simulink model "efficient_discrete_ADRC"  (R2025b)
settings: Solver=VariableStepAuto  StartTime=0.0  StopTime=20  RelTol=1e-3
values from neighbouring files (symbols this model uses):
  accelBC = nan(size(waypoints))    [quad_params.m]
  Alloc = [ kf,     kf,     kf,     kf ... (first row only)    [quad_params.m]
  Area = 2*L*Width    (= 0.072)    [quad_params.m]
  g = 9.81    [quad_params.m]
  h = [0 ... (first row only)    [Madgwick.m]    (also in quad_params.m = 0.2; umich_learning.m = x(:,1))
  h0 = Ts    (= 0.001)    [quad_params.m]
  h0_angle = Ts * 10    (= 0.01)    [quad_params.m]
  h0_h = Ts_h    (= 0.05)    [quad_params.m]
  inertia_mx = [Ixx; Iyy; Izz;]    [quad_params.m]
  init_h = 0.03    [quad_params.m]
  jerkBC = nan(size(waypoints))    [quad_params.m]
  K_alloc = Alloc \ diag([W, 1, 1, 1])    [quad_params.m]
  max_rad_s_2 = max_rad_s ^ 2    (= 4279618.17072)    [quad_params.m]
  r0_angle = 1000    [quad_params.m]
  r0_h = 1    [quad_params.m]
  r0_position = 1    [quad_params.m]
  rho_air = 1.225    [quad_params.m]
  rho_water = 1000    [quad_params.m]
  timePoints = [0, tTakeoff +      (0:nPerLoop*nLoops)*(tLoop/nPerLoop)]    [quad_params.m]
  Trot = 0.01    [quad_params.m]
  Ts = 0.001    [get_noise.m]    (also in quad_params.m; test.m = 0.002)
  Ts_h = 0.05    [quad_params.m]
  velBC = nan(size(waypoints))    [quad_params.m]
  W = 0.7 + 4*m_prop    (= 0.74)    [quad_params.m]
  waypoints = [0, x ... (first row only)    [quad_params.m]
undefined symbols (not defined in the file or in its folder): adrcD
libraries: eeGeneralControl x9, simulink x5, aerolibwind2 x1, shareduavrstlib x1
settings Model: Creator=David  LastModifiedBy=David

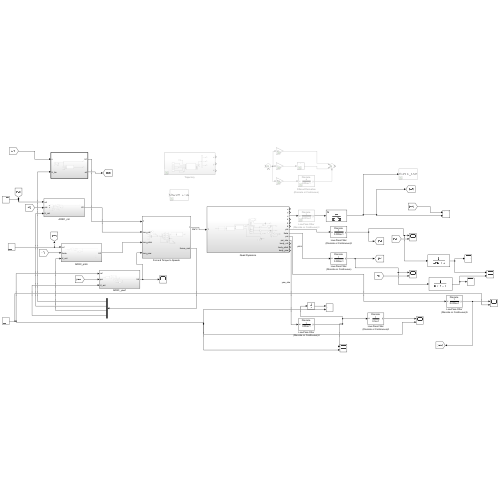
[thumbnail: Simulink's stored preview of the top-level diagram]
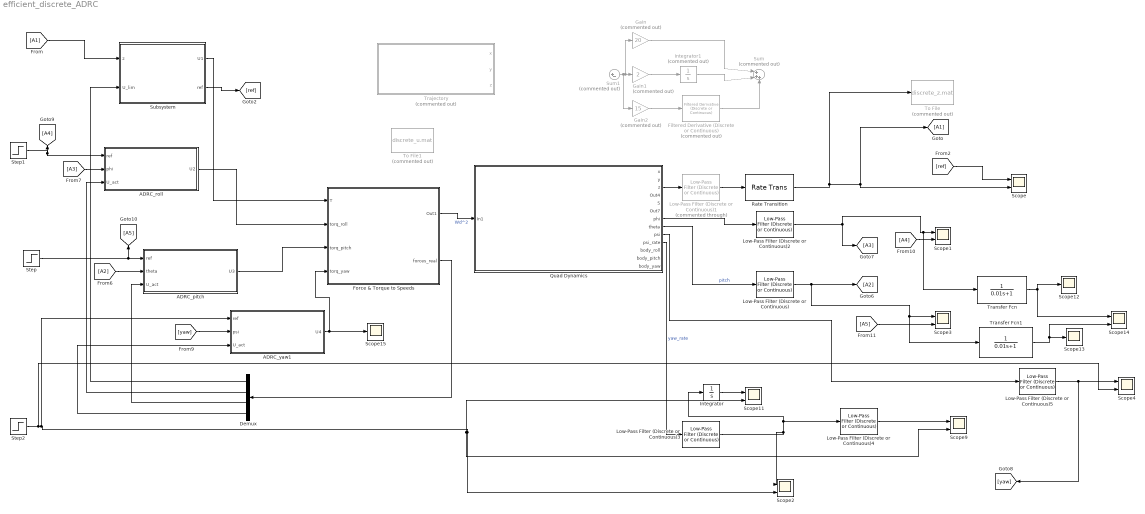
== system efficient_discrete_ADRC ==
  ADRC_pitch : Subsystem
  ADRC_roll : Subsystem
  ADRC_yaw1 : Subsystem
  Demux : Demux
  Filtered Derivative (Discrete or Continuous) : eeGeneralControl/Filtered Derivative (Discrete or Continuous)  Commented=on  K=1  T=0.05  B=inf  A=-inf  minRatio=10  init_option=Inherited from block input  x0=0  Ts=-1
      settings: LibrarySourceBlock=|
      | ee_sl_lib/General Control/Filtered Derivative
      | (Discrete or Continuous)
  Force & Torque to Speeds : Subsystem
  Gain : Gain  Commented=on  Gain=20
  Gain1 : Gain  Commented=on  Gain=2
  Gain2 : Gain  Commented=on  Gain=15
  Integrator : Integrator
  Integrator1 : Integrator  Commented=on
  Low-Pass Filter (Discrete or Continuous) : eeGeneralControl/Low-Pass Filter (Discrete or Continuous)  K=1  T=0.005  B=inf  A=-inf  init_option=Inherited from block input  x0=0  Ts=Ts
  Low-Pass Filter (Discrete or Continuous)1 : eeGeneralControl/Low-Pass Filter (Discrete or Continuous)  Commented=through  K=1  T=0.001  B=inf  A=-inf  init_option=Inherited from block input  x0=0  Ts=Ts
  Low-Pass Filter (Discrete or Continuous)2 : eeGeneralControl/Low-Pass Filter (Discrete or Continuous)  K=1  T=0.005  B=inf  A=-inf  init_option=Inherited from block input  x0=0  Ts=Ts
  Low-Pass Filter (Discrete or Continuous)3 : eeGeneralControl/Low-Pass Filter (Discrete or Continuous)  K=1  T=0.05  B=inf  A=-inf  init_option=Inherited from block input  x0=0  Ts=Ts
  Low-Pass Filter (Discrete or Continuous)4 : eeGeneralControl/Low-Pass Filter (Discrete or Continuous)  K=1  T=0.5  B=inf  A=-inf  init_option=Inherited from block input  x0=0  Ts=Ts
  Low-Pass Filter (Discrete or Continuous)5 : eeGeneralControl/Low-Pass Filter (Discrete or Continuous)  K=1  T=0.005  B=inf  A=-inf  init_option=Inherited from block input  x0=0  Ts=Ts
  Quad Dynamics : Subsystem
  Rate Transition : RateTransition  OutPortSampleTime=Ts_h
  Scope{,1..4,9,11,14} (8 alike) : Scope  NumInputPorts=2
      Scope settings: ActiveDisplayYMinimum=-0.18688766628594322  ActiveDisplayYMaximum=1.6819889965734893  DataLoggingVariableName=ScopeData2
      Scope1 settings: ActiveDisplayYMinimum=-0.13984430574300916  ActiveDisplayYMaximum=0.55327810674461919
      Scope11 settings: ActiveDisplayYMinimum=-1.1201443068824162  ActiveDisplayYMaximum=8.8240715745492686  DataLoggingVariableName=ScopeData21
      Scope14 settings: ActiveDisplayYMinimum=-0.12705190538512617  ActiveDisplayYMaximum=0.50097031332501329  DataLoggingVariableName=ScopeData29
      Scope2 settings: ActiveDisplayYMinimum=-1.0000255800633333  ActiveDisplayYMaximum=2.2551550054891538  DataLoggingVariableName=ScopeData13
      Scope3 settings: ActiveDisplayYMinimum=-1.3031757015702203  ActiveDisplayYMaximum=1.3764664599479359
      Scope4 settings: ActiveDisplayYMinimum=-0.027434331958352268  ActiveDisplayYMaximum=0.24653328293336874  DataLoggingVariableName=ScopeData4
      Scope9 settings: ActiveDisplayYMinimum=-2.6902354434565239  ActiveDisplayYMaximum=2.8491881506489021  DataLoggingVariableName=ScopeData15
  Scope12 : Scope
      settings: ActiveDisplayYMinimum=-0.051654354222600722  ActiveDisplayYMaximum=0.34551857931943891  DataLoggingVariableName=ScopeData27
  Scope13 : Scope
      settings: ActiveDisplayYMinimum=-0.043384499181721006  ActiveDisplayYMaximum=0.23881982281001995  DataLoggingVariableName=ScopeData28
  Scope15 : Scope
      settings: ActiveDisplayYMinimum=-0.42131356048161295  ActiveDisplayYMaximum=0.725418465428479  DataLoggingVariableName=ScopeData14
  Step : Step  Time=8  After=0.25  SampleTime=0
  Step1 : Step  Time=5  After=0.4  SampleTime=0
  Step2 : Step  After=0.2  SampleTime=0
  Subsystem : Subsystem  TreatAsAtomicUnit=on  SystemSampleTime=Ts_h
  Sum : Sum  Commented=on  Inputs=|+++
  Sum1 : Sum  Commented=on  Inputs=|+-
  To File : ToFile  Commented=on  Filename=discrete_z.mat  SaveFormat=Timeseries
  To File1 : ToFile  Commented=on  Filename=discrete_u.mat  SaveFormat=Timeseries
  Trajectory : Subsystem  Commented=on
  Transfer Fcn : TransferFcn  Denominator=[0.01 1]
  Transfer Fcn1 : TransferFcn  Denominator=[0.01 1]
  wires:
  Quad Dynamics/3(z) -> Low-Pass Filter (Discrete or Continuous)1/1
  [A3] -> ADRC_roll/2(phi)
  Step/1 -> ADRC_pitch/1(ref), [A5]
  Demux/2 -> ADRC_roll/3(U_act)
  Demux/4 -> ADRC_yaw1/3(U_act)
  [A5] -> Scope3/2
  [A4] -> Scope1/2
  [yaw] -> ADRC_yaw1/2(psi)
  Step1/1 -> ADRC_roll/1(ref), [A4]
  Quad Dynamics/7(phi) -> Low-Pass Filter (Discrete or Continuous)2/1
  Quad Dynamics/8(theta) -> Low-Pass Filter (Discrete or Continuous)/1  "pitch"
  Force & Torque to Speeds/1(Out1) -> Quad Dynamics/1(In1)  "Wd^2"
  Step2/1 -> Scope4/2, Scope2/2, Scope9/2, Scope11/2, ADRC_yaw1/1(ref)
  Quad Dynamics/10(psi_rate) -> Low-Pass Filter (Discrete or Continuous)3/1  "yaw_rate"
  Force & Torque to Speeds/2(forces_real) -> Demux/1
  [A2] -> ADRC_pitch/2(theta)
  Demux/3 -> ADRC_pitch/3(U_act)
  ADRC_yaw1/1(U4) -> Force & Torque to Speeds/4(torq_yaw), Scope15/1
  Integrator/1 -> Scope11/1
  Low-Pass Filter (Discrete or Continuous)1/1 -> Rate Transition/1
  Low-Pass Filter (Discrete or Continuous)2/1 -> Transfer Fcn/1, Scope1/1, [A3]
  Transfer Fcn/1 -> Scope12/1, Scope14/1
  Transfer Fcn1/1 -> Scope14/2, Scope13/1
  Low-Pass Filter (Discrete or Continuous)/1 -> Transfer Fcn1/1, Scope3/1, [A2]
  Integrator1/1 -> Sum/2
  Gain/1 -> Sum/1
  Filtered Derivative (Discrete or Continuous)/1 -> Sum/3
  Gain1/1 -> Integrator1/1
  Gain2/1 -> Filtered Derivative (Discrete or Continuous)/1
  Sum1/1 -> Gain2/1, Gain/1, Gain1/1
  [A1] -> Subsystem/1(z)
  Low-Pass Filter (Discrete or Continuous)3/1 -> Integrator/1, Low-Pass Filter (Discrete or Continuous)4/1, Scope2/1
  Low-Pass Filter (Discrete or Continuous)4/1 -> Scope9/1
  ADRC_roll/1(U2) -> Force & Torque to Speeds/2(torq_roll)
  ADRC_pitch/1(U3) -> Force & Torque to Speeds/3(torq_pitch)
  [ref] -> Scope/1
  Rate Transition/1 -> To File/1, [A1], Scope/2
  Quad Dynamics/9(psi) -> Low-Pass Filter (Discrete or Continuous)5/1
  Low-Pass Filter (Discrete or Continuous)5/1 -> [yaw], Scope4/1
  Demux/1 -> Subsystem/2(U_lim)
  Subsystem/2(ref) -> [ref]
  Subsystem/1(U1) -> Force & Torque to Speeds/1(T)

== system efficient_discrete_ADRC/ADRC_pitch ==
  ref : Inport
  theta : Inport  Port=2
  U_act : Inport  Port=3
  Constant : Constant  Value=adrcD.pitch.b0
  Divide : Product  Inputs=*/
  Filtered Derivative (Discrete or Continuous) : eeGeneralControl/Filtered Derivative (Discrete or Continuous)  K=1  T=1*Ts  B=inf  A=-inf  minRatio=1  init_option=Inherited from block input  x0=0  Ts=Ts
      settings: LibrarySourceBlock=|
      | ee_sl_lib/General Control/Filtered Derivative
      | (Discrete or Continuous)
  Gain : Gain  Gain=adrcD.pitch.k1
  Gain2 : Gain  Gain=adrcD.pitch.k2
  Scope1 : Scope
      settings: DataLoggingVariableName=ScopeData18
  Scope2 : Scope
      settings: DataLoggingVariableName=ScopeData19
  Sum1 : Sum  Inputs=|++
  Sum2 : Sum  Inputs=|++
  adrcD : Subsystem
  U3 : Outport
  wires:
  ref/1 -> Gain/1, Filtered Derivative (Discrete or Continuous)/1
  Sum1/1 -> U3/1
  Divide/1 -> Sum1/1
  Constant/1 -> Divide/2
  Gain/1 -> Sum2/1
  Filtered Derivative (Discrete or Continuous)/1 -> Gain2/1
  Gain2/1 -> Sum2/2
  Sum2/1 -> Divide/1
  adrcD/1(U) -> Sum1/2
  theta/1 -> adrcD/2(y)
  U_act/1 -> adrcD/1(U_act)

== system efficient_discrete_ADRC/ADRC_roll ==
  ref : Inport
  phi : Inport  Port=2
  U_act : Inport  Port=3
  Constant : Constant  Value=adrcD.roll.b0
  Divide : Product  Inputs=*/
  Filtered Derivative (Discrete or Continuous) : eeGeneralControl/Filtered Derivative (Discrete or Continuous)  K=1  T=1*Ts  B=inf  A=-inf  minRatio=1  init_option=Inherited from block input  x0=0  Ts=Ts
      settings: LibrarySourceBlock=|
      | ee_sl_lib/General Control/Filtered Derivative
      | (Discrete or Continuous)
  Gain : Gain  Gain=adrcD.roll.k1
  Gain2 : Gain  Gain=adrcD.roll.k2
  Scope : Scope  NumInputPorts=2
      settings: ActiveDisplayYMinimum=-0.12874999999999998  ActiveDisplayYMaximum=1.15875  DataLoggingVariableName=ScopeData3
  Scope1 : Scope  NumInputPorts=2
      settings: ActiveDisplayYMinimum=-49.999999999999986  ActiveDisplayYMaximum=450  DataLoggingVariableName=ScopeData20
  Sum1 : Sum  Inputs=|++
  Sum2 : Sum  Inputs=|++
  TD1 : Subsystem
  adrcD : Subsystem
  U2 : Outport
  wires:
  ref/1 -> Filtered Derivative (Discrete or Continuous)/1, Scope/2, TD1/1(v)
  Sum1/1 -> U2/1
  Divide/1 -> Sum1/1
  Constant/1 -> Divide/2
  Gain/1 -> Sum2/1
  TD1/2(dref) -> Scope/1, Scope1/2, Gain2/1
  Gain2/1 -> Sum2/2
  Sum2/1 -> Divide/1
  adrcD/1(U) -> Sum1/2
  U_act/1 -> adrcD/1(U_act)
  phi/1 -> adrcD/2(y)
  TD1/1(ref) -> Gain/1
  Filtered Derivative (Discrete or Continuous)/1 -> Scope1/1

== system efficient_discrete_ADRC/ADRC_yaw1 ==
  ref : Inport
  psi : Inport  Port=2
  U_act : Inport  Port=3
  Constant : Constant  Value=adrcD.yaw.b0
  Divide : Product  Inputs=*/
  Gain : Gain  Gain=adrcD.yaw.k1
  Gain2 : Gain  Gain=adrcD.yaw.k2
  Scope : Scope
      settings: DataLoggingVariableName=ScopeData23
  Sum1 : Sum  Inputs=|++
  Sum2 : Sum  Inputs=|++
  TD1 : Subsystem
  adrcD : Subsystem
  U4 : Outport
  wires:
  Sum1/1 -> U4/1
  Divide/1 -> Sum1/1
  Constant/1 -> Divide/2
  ref/1 -> TD1/1(v)
  TD1/1(ref) -> Gain/1
  TD1/2(dref) -> Gain2/1
  Gain/1 -> Sum2/1
  Gain2/1 -> Sum2/2
  Sum2/1 -> Scope/1, Divide/1
  adrcD/1(U) -> Sum1/2
  U_act/1 -> adrcD/1(U_act)
  psi/1 -> adrcD/2(y)

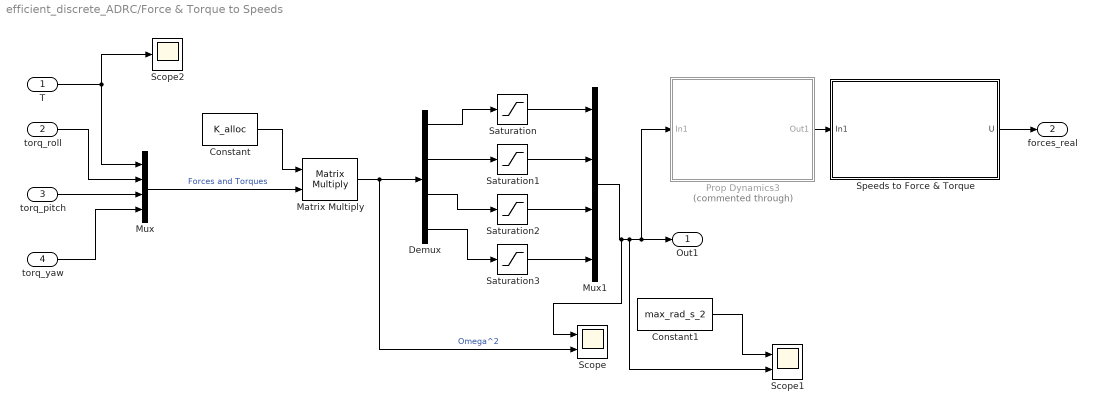
== system efficient_discrete_ADRC/Force & Torque to Speeds ==
  T : Inport
  torq_roll : Inport  Port=2
  torq_pitch : Inport  Port=3
  torq_yaw : Inport  Port=4
  Constant : Constant  Value=K_alloc
  Constant1 : Constant  Value=max_rad_s_2
  Demux : Demux
  Matrix Multiply : Product  Multiplication=Matrix(*)
  Mux : Mux
  Mux1 : Mux
  Prop Dynamics3 : Subsystem  Commented=through
  Saturation{,1..3} (4 alike) : Saturate  UpperLimit=max_rad_s_2  LowerLimit=0
  Scope : Scope  NumInputPorts=2
      settings: ActiveDisplayYMinimum=-2.4803736586129647E+6  ActiveDisplayYMaximum=5.5202696731347125E+6  DataLoggingVariableName=ScopeData11
  Scope1 : Scope  NumInputPorts=2
      settings: ActiveDisplayYMinimum=-534952.27133938007  ActiveDisplayYMaximum=4.8145704420544216E+6  DataLoggingVariableName=ScopeData25
  Scope2 : Scope
      settings: ActiveDisplayYMinimum=-22.315254964417129  ActiveDisplayYMaximum=34.792796764645914  DataLoggingVariableName=ScopeData9
  Speeds to Force & Torque : Subsystem
  Out1 : Outport
  forces_real : Outport  Port=2
  wires:
  Matrix Multiply/1 -> Scope/2, Demux/1  "Omega^2"
  torq_yaw/1 -> Mux/4
  torq_pitch/1 -> Mux/3
  torq_roll/1 -> Mux/2
  T/1 -> Mux/1, Scope2/1
  Constant/1 -> Matrix Multiply/1
  Mux/1 -> Matrix Multiply/2  "Forces and Torques"
  Saturation3/1 -> Mux1/4
  Demux/4 -> Saturation3/1
  Demux/2 -> Saturation1/1
  Demux/1 -> Saturation/1
  Demux/3 -> Saturation2/1
  Saturation1/1 -> Mux1/2
  Saturation/1 -> Mux1/1
  Saturation2/1 -> Mux1/3
  Mux1/1 -> Scope/1, Scope1/2, Prop Dynamics3/1(In1), Out1/1
  Speeds to Force & Torque/1(U) -> forces_real/1
  Prop Dynamics3/1(Out1) -> Speeds to Force & Torque/1(In1)
  Constant1/1 -> Scope1/1

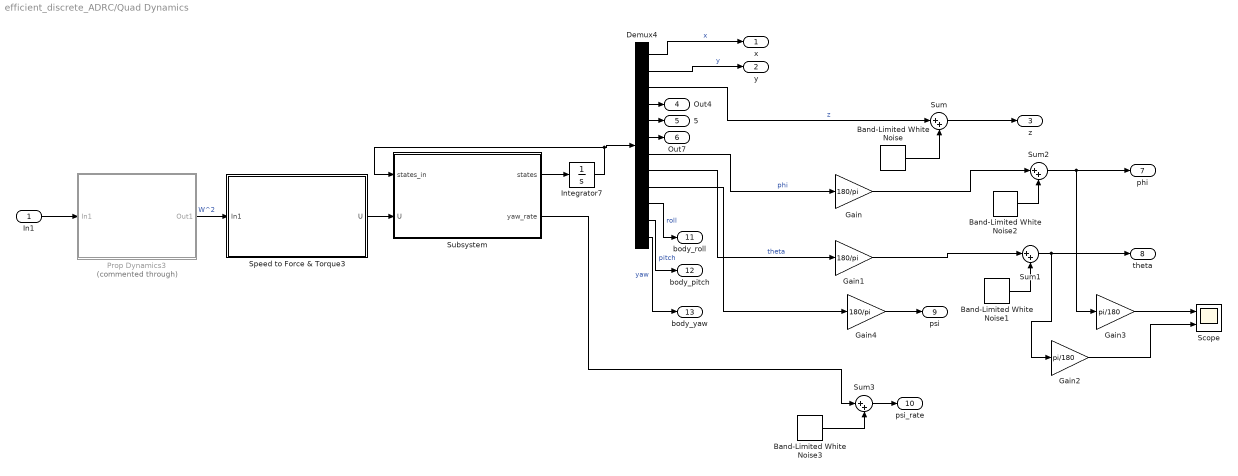
== system efficient_discrete_ADRC/Quad Dynamics ==
  In1 : Inport
  Band-Limited White Noise : simulink/Sources/Band-Limited White Noise  Cov=[2.6540e-06]  Ts=Ts_h  seed=[23341]
  Band-Limited White Noise1 : simulink/Sources/Band-Limited White Noise  Cov=[2e-6]  Ts=0.001  seed=[23342]
  Band-Limited White Noise2 : simulink/Sources/Band-Limited White Noise  Cov=[2e-6]  Ts=0.001  seed=[23341]
  Band-Limited White Noise3 : simulink/Sources/Band-Limited White Noise  Cov=[3.7430331138e-5]  Ts=0.001  seed=[23343]
  Demux4 : Demux  Outputs=12
  Gain : Gain  Gain=180/pi
  Gain1 : Gain  Gain=180/pi
  Gain2 : Gain  Gain=pi/180
  Gain3 : Gain  Gain=pi/180
  Gain4 : Gain  Gain=180/pi
  Integrator7 : Integrator  InitialCondition=zeros(12,1)
  Prop Dynamics3 : Subsystem  Commented=through
  Scope : Scope  NumInputPorts=2
      settings: ActiveDisplayYMinimum=-1  ActiveDisplayYMaximum=1  DataLoggingVariableName=ScopeData16
  Speed to Force & Torque3 : Subsystem
  Subsystem : Subsystem
  Sum{,1..3} (4 alike) : Sum  Inputs=|++
  x : Outport
  y : Outport  Port=2
  z : Outport  Port=3
  Out4 : Outport  Port=4
  5 : Outport  Port=5
  Out7 : Outport  Port=6
  phi : Outport  Port=7
  theta : Outport  Port=8
  psi : Outport  Port=9
  psi_rate : Outport  Port=10
  body_roll : Outport  Port=11
  body_pitch : Outport  Port=12
  body_yaw : Outport  Port=13
  wires:
  Demux4/2 -> y/1  "y"
  Prop Dynamics3/1(Out1) -> Speed to Force & Torque3/1(In1)  "W^2"
  Demux4/1 -> x/1  "x"
  Subsystem/1(states) -> Integrator7/1
  Speed to Force & Torque3/1(U) -> Subsystem/2(U)
  Integrator7/1 -> Demux4/1, Subsystem/1(states_in)
  Demux4/10 -> body_roll/1  "roll"
  Demux4/7 -> Gain/1  "phi"
  Demux4/3 -> Sum/1  "z"
  Demux4/8 -> Gain1/1  "theta"
  Demux4/11 -> body_pitch/1  "pitch"
  Demux4/12 -> body_yaw/1  "yaw"
  Demux4/6 -> Out7/1
  Demux4/5 -> 5/1
  Demux4/4 -> Out4/1
  In1/1 -> Prop Dynamics3/1(In1)
  Subsystem/2(yaw_rate) -> Sum3/1
  Sum/1 -> z/1
  Band-Limited White Noise/1 -> Sum/2
  Band-Limited White Noise1/1 -> Sum1/2
  Sum1/1 -> Gain2/1, theta/1
  Band-Limited White Noise2/1 -> Sum2/2
  Sum2/1 -> Gain3/1, phi/1
  Band-Limited White Noise3/1 -> Sum3/2
  Sum3/1 -> psi_rate/1
  Gain/1 -> Sum2/1
  Gain1/1 -> Sum1/1
  Gain3/1 -> Scope/1
  Gain2/1 -> Scope/2
  Demux4/9 -> Gain4/1
  Gain4/1 -> psi/1

== system efficient_discrete_ADRC/Subsystem ==
  z : Inport
  U_lim : Inport  Port=2
  ADRC_z : Subsystem
  Constant4 : Constant  Value=init_h
  Step3 : Step  Time=2
  Sum7 : Sum  Inputs=|++
  U1 : Outport
  ref : Outport  Port=2
  wires:
  Sum7/1 -> ADRC_z/1(ref), ref/1  "ref"
  Step3/1 -> Sum7/1  "v"
  U_lim/1 -> ADRC_z/3(U_lim)
  ADRC_z/1(U1) -> U1/1
  Constant4/1 -> Sum7/2
  z/1 -> ADRC_z/2(z)

== system efficient_discrete_ADRC/Trajectory ==
  Constant1 : Constant  Value=timePoints
  Constant2 : Constant  Value=waypoints
  Constant3 : Constant  Value=velBC
  Constant4 : Constant  Value=accelBC
  Constant5 : Constant  Value=jerkBC
  Demux : Demux  Outputs=3
  Minimum Jerk Polynomial Trajectory : shareduavrstlib/Minimum Jerk Polynomial Trajectory  ShowBCInputPort=on  ShowPolynomialCoefs=off  ShowStatusOutputPort=off  TimeAllocation=off  TimeWeight=100  MinSegmentTime=0.1  MaxSegmentTime=1  MaxIteration=1500  MaxTime=10  SimulateUsing=Interpreted execution
  Ramp : simulink/Sources/Ramp  slope=1  start=0  InitialOutput=0
  Scope8 : Scope
      settings: ActiveDisplayYMinimum=-1  ActiveDisplayYMaximum=1  DataLoggingVariableName=ScopeData17
  Terminator : Terminator
  Terminator1 : Terminator
  Terminator2 : Terminator
  x : Outport
  y : Outport  Port=2
  z : Outport  Port=3
  wires:
  Minimum Jerk Polynomial Trajectory/4 -> Terminator1/1
  Minimum Jerk Polynomial Trajectory/2 -> Scope8/1
  Constant3/1 -> Minimum Jerk Polynomial Trajectory/4
  Constant2/1 -> Minimum Jerk Polynomial Trajectory/2
  Ramp/1 -> Minimum Jerk Polynomial Trajectory/1
  Minimum Jerk Polynomial Trajectory/3 -> Terminator/1
  Constant5/1 -> Minimum Jerk Polynomial Trajectory/6
  Constant4/1 -> Minimum Jerk Polynomial Trajectory/5
  Minimum Jerk Polynomial Trajectory/5 -> Terminator2/1
  Constant1/1 -> Minimum Jerk Polynomial Trajectory/3
  Minimum Jerk Polynomial Trajectory/1 -> Demux/1  "height"
  Demux/1 -> x/1
  Demux/2 -> y/1
  Demux/3 -> z/1

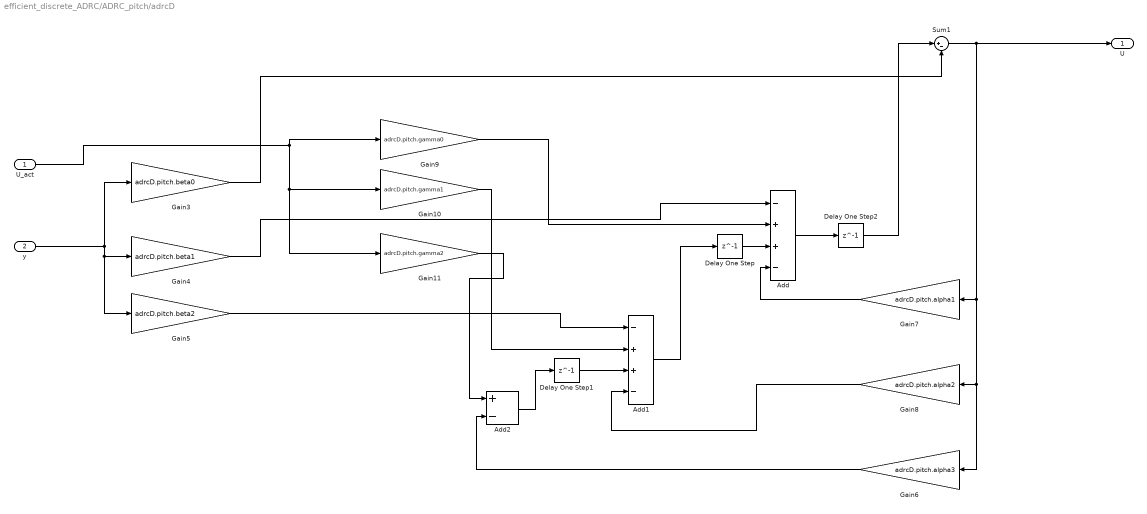
== system efficient_discrete_ADRC/ADRC_pitch/adrcD ==
  U_act : Inport
  y : Inport  Port=2
  Add : Sum  Inputs=-++-
  Add1 : Sum  Inputs=-++-
  Add2 : Sum  Inputs=+-
  Delay One Step : Delay  DelayLength=1  SampleTime=Ts
  Delay One Step1 : Delay  DelayLength=1  SampleTime=Ts
  Delay One Step2 : Delay  DelayLength=1  SampleTime=Ts
  Gain10 : Gain  Gain=adrcD.pitch.gamma1
  Gain11 : Gain  Gain=adrcD.pitch.gamma2
  Gain3 : Gain  Gain=adrcD.pitch.beta0
  Gain4 : Gain  Gain=adrcD.pitch.beta1
  Gain5 : Gain  Gain=adrcD.pitch.beta2
  Gain6 : Gain  Gain=adrcD.pitch.alpha3
  Gain7 : Gain  Gain=adrcD.pitch.alpha1
  Gain8 : Gain  Gain=adrcD.pitch.alpha2
  Gain9 : Gain  Gain=adrcD.pitch.gamma0
  Sum1 : Sum  Inputs=|+-
  U : Outport
  wires:
  Gain4/1 -> Add/1
  Gain8/1 -> Add1/4
  Add2/1 -> Delay One Step1/1
  y/1 -> Gain5/1, Gain4/1, Gain3/1
  U_act/1 -> Gain9/1, Gain11/1, Gain10/1
  Gain7/1 -> Add/4
  Gain11/1 -> Add2/1
  Gain3/1 -> Sum1/2
  Sum1/1 -> U/1, Gain6/1, Gain8/1, Gain7/1
  Add1/1 -> Delay One Step/1
  Gain5/1 -> Add1/1
  Gain10/1 -> Add1/2
  Add/1 -> Delay One Step2/1
  Gain9/1 -> Add/2
  Delay One Step1/1 -> Add1/3
  Delay One Step2/1 -> Sum1/1
  Gain6/1 -> Add2/2
  Delay One Step/1 -> Add/3

== system efficient_discrete_ADRC/ADRC_roll/TD1 ==
  v : Inport
  Constant11 : Constant  Value=r0_angle
  Constant12 : Constant  Value=h0_angle
  Delay One Step : Delay  DelayLength=1  SampleTime=Ts
  Delay One Step1 : Delay  DelayLength=1  SampleTime=Ts
  Gain3 : Gain  Gain=Ts
  Gain4 : Gain  Gain=Ts
  Sum1 : Sum  Inputs=|++
  Sum6 : Sum  Inputs=|++
  Sum7 : Sum  Inputs=|+-
  fhan : MATLAB Function  TreatAsAtomicUnit=on
  ref : Outport
  dref : Outport  Port=2
  wires:
  v/1 -> Sum7/2
  Constant12/1 -> fhan/4(h0)
  Sum7/1 -> fhan/1(e)
  Constant11/1 -> fhan/3(r0)
  Delay One Step1/1 -> fhan/2(v2), Sum6/2, Gain4/1  "v2(k)"
  Gain4/1 -> Sum1/2
  Sum1/1 -> ref/1, Delay One Step/1  "v1(k+1)"
  Sum6/1 -> dref/1, Delay One Step1/1  "v2(k+1)"
  Gain3/1 -> Sum6/1
  Delay One Step/1 -> Sum1/1, Sum7/1  "v1"
  fhan/1(u) -> Gain3/1

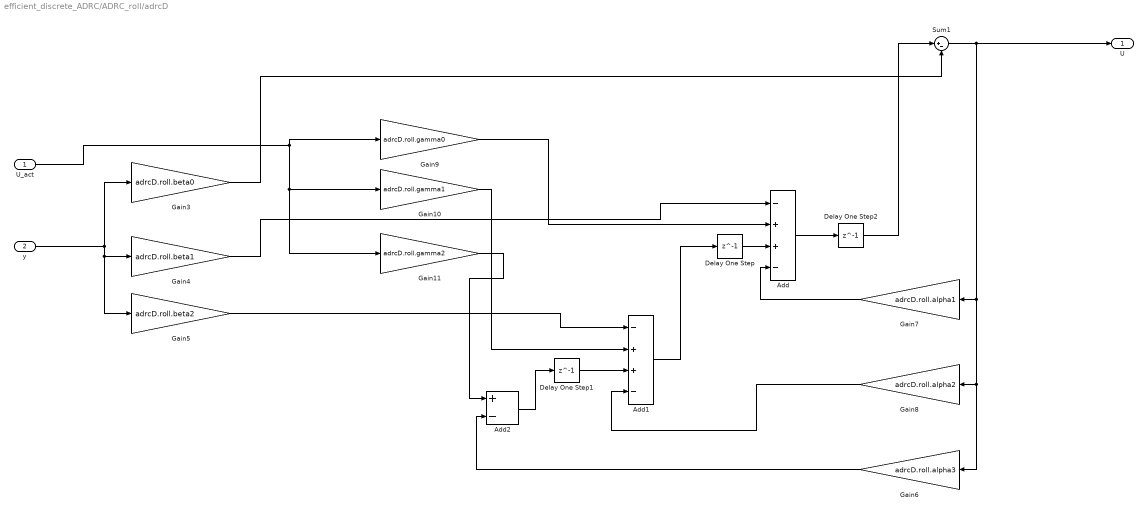
== system efficient_discrete_ADRC/ADRC_roll/adrcD ==
  U_act : Inport
  y : Inport  Port=2
  Add : Sum  Inputs=-++-
  Add1 : Sum  Inputs=-++-
  Add2 : Sum  Inputs=+-
  Delay One Step : Delay  DelayLength=1  SampleTime=Ts
  Delay One Step1 : Delay  DelayLength=1  SampleTime=Ts
  Delay One Step2 : Delay  DelayLength=1  SampleTime=Ts
  Gain10 : Gain  Gain=adrcD.roll.gamma1
  Gain11 : Gain  Gain=adrcD.roll.gamma2
  Gain3 : Gain  Gain=adrcD.roll.beta0
  Gain4 : Gain  Gain=adrcD.roll.beta1
  Gain5 : Gain  Gain=adrcD.roll.beta2
  Gain6 : Gain  Gain=adrcD.roll.alpha3
  Gain7 : Gain  Gain=adrcD.roll.alpha1
  Gain8 : Gain  Gain=adrcD.roll.alpha2
  Gain9 : Gain  Gain=adrcD.roll.gamma0
  Sum1 : Sum  Inputs=|+-
  U : Outport
  wires:
  Gain4/1 -> Add/1
  Gain8/1 -> Add1/4
  Add2/1 -> Delay One Step1/1
  y/1 -> Gain5/1, Gain4/1, Gain3/1
  U_act/1 -> Gain9/1, Gain11/1, Gain10/1
  Gain7/1 -> Add/4
  Gain11/1 -> Add2/1
  Gain3/1 -> Sum1/2
  Sum1/1 -> U/1, Gain6/1, Gain8/1, Gain7/1
  Add1/1 -> Delay One Step/1
  Gain5/1 -> Add1/1
  Gain10/1 -> Add1/2
  Add/1 -> Delay One Step2/1
  Gain9/1 -> Add/2
  Delay One Step1/1 -> Add1/3
  Delay One Step2/1 -> Sum1/1
  Gain6/1 -> Add2/2
  Delay One Step/1 -> Add/3

== system efficient_discrete_ADRC/ADRC_yaw1/TD1 ==
  v : Inport
  Constant11 : Constant  Value=r0_position
  Constant12 : Constant  Value=h0
  Delay One Step : Delay  DelayLength=1  SampleTime=Ts
  Delay One Step1 : Delay  DelayLength=1  SampleTime=Ts
  Gain3 : Gain  Gain=Ts
  Gain4 : Gain  Gain=Ts
  Sum1 : Sum  Inputs=|++
  Sum6 : Sum  Inputs=|++
  Sum7 : Sum  Inputs=|+-
  fhan : MATLAB Function  TreatAsAtomicUnit=on
  ref : Outport
  dref : Outport  Port=2
  wires:
  v/1 -> Sum7/2
  Constant12/1 -> fhan/4(h0)
  Sum7/1 -> fhan/1(e)
  Constant11/1 -> fhan/3(r0)
  Delay One Step1/1 -> fhan/2(v2), Sum6/2, Gain4/1  "v2(k)"
  Gain4/1 -> Sum1/2
  Sum1/1 -> ref/1, Delay One Step/1  "v1(k+1)"
  Sum6/1 -> dref/1, Delay One Step1/1  "v2(k+1)"
  Gain3/1 -> Sum6/1
  Delay One Step/1 -> Sum1/1, Sum7/1  "v1"
  fhan/1(u) -> Gain3/1

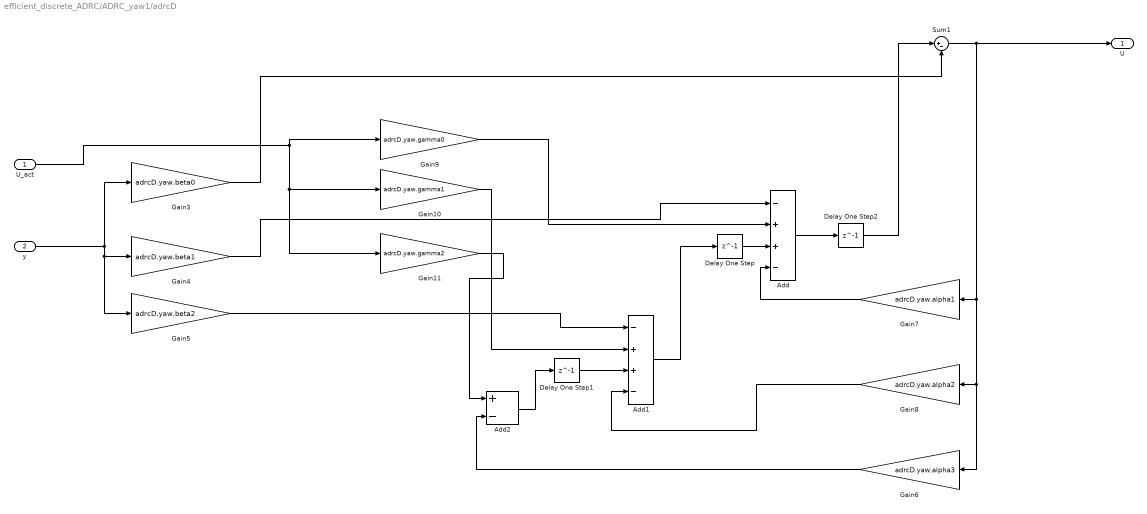
== system efficient_discrete_ADRC/ADRC_yaw1/adrcD ==
  U_act : Inport
  y : Inport  Port=2
  Add : Sum  Inputs=-++-
  Add1 : Sum  Inputs=-++-
  Add2 : Sum  Inputs=+-
  Delay One Step : Delay  DelayLength=1  SampleTime=Ts
  Delay One Step1 : Delay  DelayLength=1  SampleTime=Ts
  Delay One Step2 : Delay  DelayLength=1  SampleTime=Ts
  Gain10 : Gain  Gain=adrcD.yaw.gamma1
  Gain11 : Gain  Gain=adrcD.yaw.gamma2
  Gain3 : Gain  Gain=adrcD.yaw.beta0
  Gain4 : Gain  Gain=adrcD.yaw.beta1
  Gain5 : Gain  Gain=adrcD.yaw.beta2
  Gain6 : Gain  Gain=adrcD.yaw.alpha3
  Gain7 : Gain  Gain=adrcD.yaw.alpha1
  Gain8 : Gain  Gain=adrcD.yaw.alpha2
  Gain9 : Gain  Gain=adrcD.yaw.gamma0
  Sum1 : Sum  Inputs=|+-
  U : Outport
  wires:
  Gain4/1 -> Add/1
  Gain8/1 -> Add1/4
  Add2/1 -> Delay One Step1/1
  y/1 -> Gain5/1, Gain4/1, Gain3/1
  U_act/1 -> Gain9/1, Gain11/1, Gain10/1
  Gain7/1 -> Add/4
  Gain11/1 -> Add2/1
  Gain3/1 -> Sum1/2
  Sum1/1 -> U/1, Gain6/1, Gain8/1, Gain7/1
  Add1/1 -> Delay One Step/1
  Gain5/1 -> Add1/1
  Gain10/1 -> Add1/2
  Add/1 -> Delay One Step2/1
  Gain9/1 -> Add/2
  Delay One Step1/1 -> Add1/3
  Delay One Step2/1 -> Sum1/1
  Gain6/1 -> Add2/2
  Delay One Step/1 -> Add/3

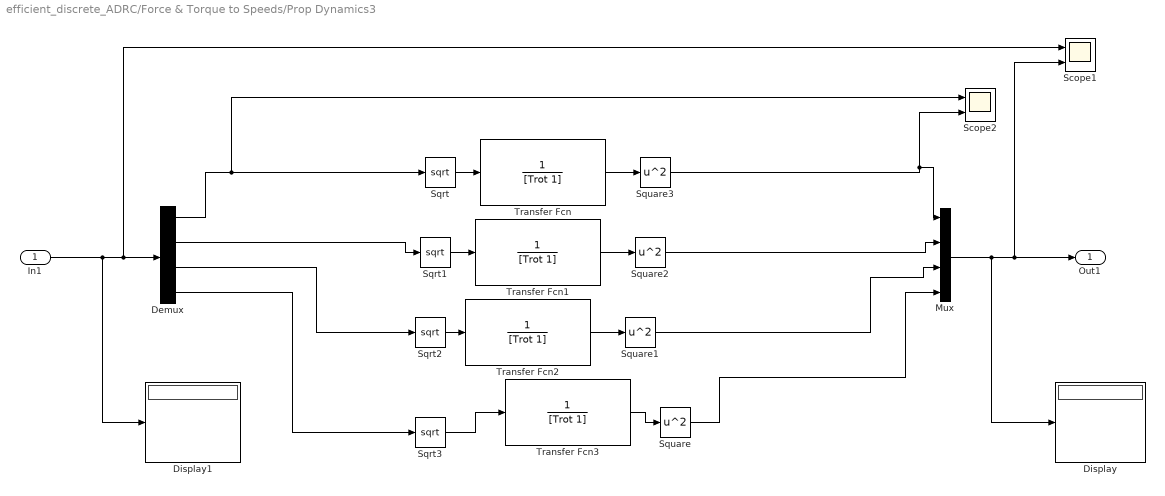
== system efficient_discrete_ADRC/Force & Torque to Speeds/Prop Dynamics3 ==
  In1 : Inport
  Demux : Demux
  Display : Display
  Display1 : Display
  Mux : Mux
  Scope1 : Scope  NumInputPorts=2
      settings: ActiveDisplayYMinimum=112181.7837613984  ActiveDisplayYMaximum=826252.36344831332  DataLoggingVariableName=ScopeData22
  Scope2 : Scope  NumInputPorts=2
      settings: ActiveDisplayYMinimum=474145.79333634069  ActiveDisplayYMaximum=566090.11578068486  DataLoggingVariableName=ScopeData26
  Sqrt{,1..3} (4 alike) : Sqrt
  Square{,1..3} (4 alike) : Math  Operator=square
  Transfer Fcn{,1..3} (4 alike) : TransferFcn  Denominator=[Trot 1]
  Out1 : Outport
  wires:
  Square/1 -> Mux/4
  Demux/4 -> Sqrt3/1
  Demux/3 -> Sqrt2/1
  Demux/2 -> Sqrt1/1
  Demux/1 -> Sqrt/1, Scope2/1
  Sqrt3/1 -> Transfer Fcn3/1
  Sqrt2/1 -> Transfer Fcn2/1
  Sqrt1/1 -> Transfer Fcn1/1
  Sqrt/1 -> Transfer Fcn/1
  Transfer Fcn3/1 -> Square/1
  Transfer Fcn2/1 -> Square1/1
  Transfer Fcn/1 -> Square3/1
  Transfer Fcn1/1 -> Square2/1
  Mux/1 -> Scope1/2, Out1/1, Display/1
  In1/1 -> Scope1/1, Demux/1, Display1/1
  Square3/1 -> Scope2/2, Mux/1
  Square2/1 -> Mux/2
  Square1/1 -> Mux/3

== system efficient_discrete_ADRC/Force & Torque to Speeds/Speeds to Force & Torque ==
  In1 : Inport
  Constant1 : Constant  Value=Alloc
  Matrix Multiply1 : Product  Multiplication=Matrix(*)
  U : Outport
  wires:
  Constant1/1 -> Matrix Multiply1/1
  Matrix Multiply1/1 -> U/1
  In1/1 -> Matrix Multiply1/2  "Omega^2"

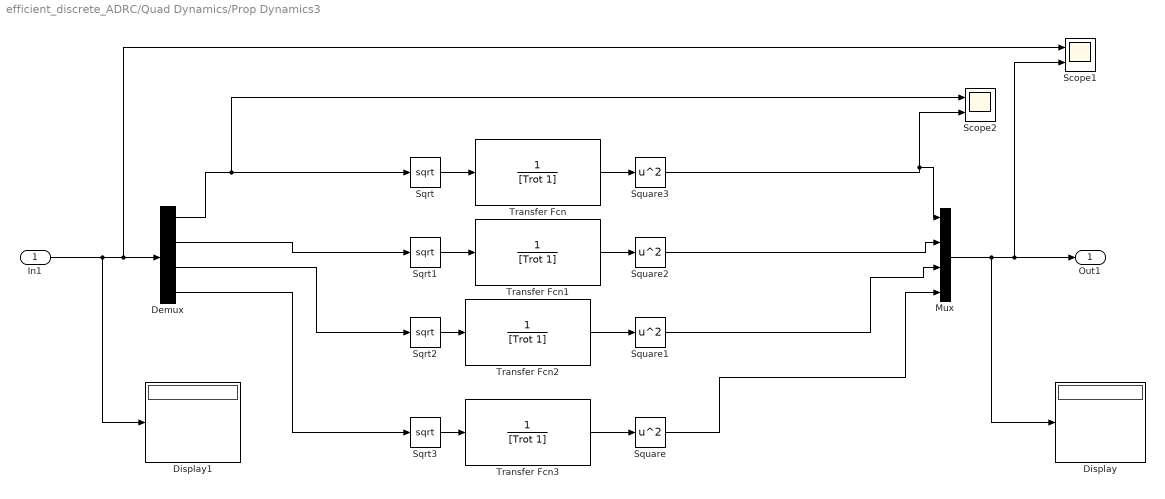
== system efficient_discrete_ADRC/Quad Dynamics/Prop Dynamics3 ==
  In1 : Inport
  Demux : Demux
  Display : Display
  Display1 : Display
  Mux : Mux
  Scope1 : Scope  NumInputPorts=2
      settings: ActiveDisplayYMinimum=-75977.2512965213  ActiveDisplayYMaximum=683795.26166869176  DataLoggingVariableName=ScopeData22
  Scope2 : Scope  NumInputPorts=2
      settings: ActiveDisplayYMinimum=-75859.286983978411  ActiveDisplayYMaximum=682733.58285580587  DataLoggingVariableName=ScopeData26
  Sqrt{,1..3} (4 alike) : Sqrt
  Square{,1..3} (4 alike) : Math  Operator=square
  Transfer Fcn{,1..3} (4 alike) : TransferFcn  Denominator=[Trot 1]
  Out1 : Outport
  wires:
  Square/1 -> Mux/4
  Demux/4 -> Sqrt3/1
  Demux/3 -> Sqrt2/1
  Demux/2 -> Sqrt1/1
  Demux/1 -> Sqrt/1, Scope2/1
  Sqrt3/1 -> Transfer Fcn3/1
  Sqrt2/1 -> Transfer Fcn2/1
  Sqrt1/1 -> Transfer Fcn1/1
  Sqrt/1 -> Transfer Fcn/1
  Transfer Fcn3/1 -> Square/1
  Transfer Fcn2/1 -> Square1/1
  Transfer Fcn/1 -> Square3/1
  Transfer Fcn1/1 -> Square2/1
  Mux/1 -> Scope1/2, Out1/1, Display/1
  In1/1 -> Scope1/1, Demux/1, Display1/1
  Square3/1 -> Scope2/2, Mux/1
  Square2/1 -> Mux/2
  Square1/1 -> Mux/3

== system efficient_discrete_ADRC/Quad Dynamics/Speed to Force & Torque3 ==
  In1 : Inport
  Constant1 : Constant  Value=Alloc
  Matrix Multiply1 : Product  Multiplication=Matrix(*)
  U : Outport
  wires:
  Constant1/1 -> Matrix Multiply1/1
  Matrix Multiply1/1 -> U/1
  In1/1 -> Matrix Multiply1/2  "Omega^2"

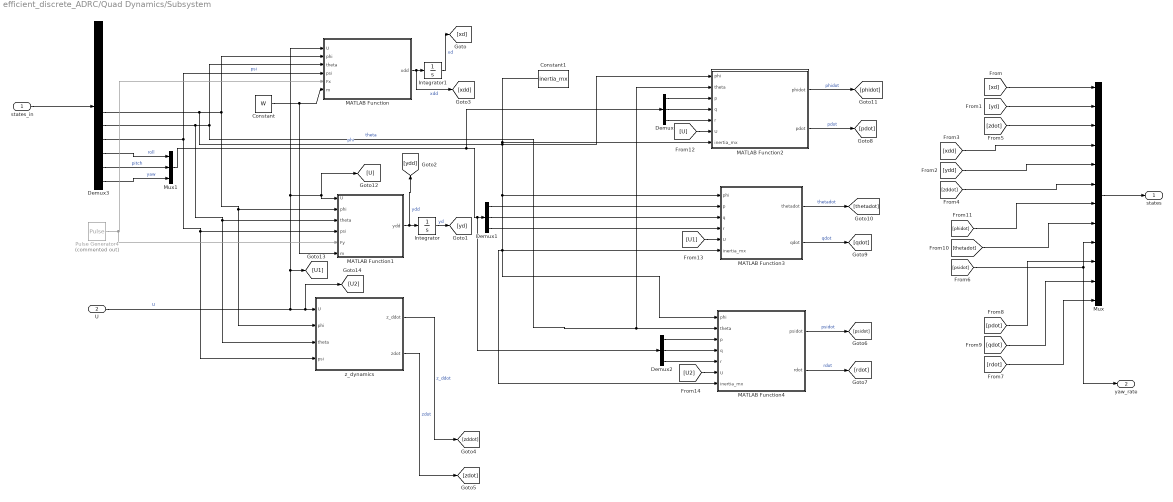
== system efficient_discrete_ADRC/Quad Dynamics/Subsystem ==
  states_in : Inport
  U : Inport  Port=2
  Constant : Constant  Value=W
  Constant1 : Constant  Value=inertia_mx
  Demux : Demux  Outputs=3
  Demux1 : Demux  Outputs=3
  Demux2 : Demux  Outputs=3
  Demux3 : Demux  Outputs=12
  Integrator : Integrator
  Integrator1 : Integrator
  MATLAB Function : MATLAB Function  TreatAsAtomicUnit=on
  MATLAB Function1 : MATLAB Function  TreatAsAtomicUnit=on
  MATLAB Function2 : MATLAB Function  TreatAsAtomicUnit=on
  MATLAB Function3 : MATLAB Function  TreatAsAtomicUnit=on
  MATLAB Function4 : MATLAB Function  TreatAsAtomicUnit=on
  Mux : Mux  Inputs=12
  Mux1 : Mux  Inputs=3
  Pulse Generator4 : DiscretePulseGenerator  Commented=on  PulseType=Time based  Amplitude=0.1  Period=5  PulseWidth=30  PhaseDelay=6
  z_dynamics : Subsystem
  states : Outport
  yaw_rate : Outport  Port=2
  wires:
  MATLAB Function/1(xdd) -> [xdd], Integrator1/1  "xdd"
  MATLAB Function1/1(ydd) -> [ydd], Integrator/1  "ydd"
  Mux/1 -> states/1
  states_in/1 -> Demux3/1
  U/1 -> [U2], z_dynamics/1(U), MATLAB Function/1(U), [U], MATLAB Function1/1(U), [U1]  "U"
  Demux3/7 -> MATLAB Function3/1(phi), MATLAB Function4/1(phi), MATLAB Function2/1(phi), MATLAB Function/2(phi), z_dynamics/2(phi), MATLAB Function1/2(phi)  "phi"
  Demux3/8 -> z_dynamics/3(theta), MATLAB Function1/3(theta), MATLAB Function2/2(theta), MATLAB Function4/2(theta), MATLAB Function/3(theta)  "theta"
  Demux3/9 -> z_dynamics/4(psi), MATLAB Function1/4(psi), MATLAB Function/4(psi)  "psi"
  Constant/1 -> MATLAB Function/6(m), MATLAB Function1/6(m)
  Constant1/1 -> MATLAB Function4/7(inertia_mx), MATLAB Function3/6(inertia_mx), MATLAB Function2/7(inertia_mx)
  Demux3/11 -> Mux1/2  "pitch"
  Demux3/12 -> Mux1/3  "yaw"
  Demux3/10 -> Mux1/1  "roll"
  Mux1/1 -> Demux/1, Demux2/1, Demux1/1
  Demux1/1 -> MATLAB Function3/2(p)
  Demux1/2 -> MATLAB Function3/3(q)
  Demux1/3 -> MATLAB Function3/4(r)
  Demux2/1 -> MATLAB Function4/3(p)
  Demux2/2 -> MATLAB Function4/4(q)
  Demux2/3 -> MATLAB Function4/5(r)
  Demux/1 -> MATLAB Function2/3(p)
  Demux/2 -> MATLAB Function2/4(q)
  Demux/3 -> MATLAB Function2/5(r)
  Integrator1/1 -> [xd]  "xd"
  [xd] -> Mux/1
  Integrator/1 -> [yd]  "yd"
  [yd] -> Mux/2
  [ydd] -> Mux/5
  [xdd] -> Mux/4
  z_dynamics/1(z_ddot) -> [zddot]  "z_ddot"
  [zddot] -> Mux/6
  z_dynamics/2(zdot) -> [zdot]  "zdot"
  [zdot] -> Mux/3
  MATLAB Function4/1(psidot) -> [psidot]  "psidot"
  [psidot] -> Mux/9, yaw_rate/1
  MATLAB Function4/2(rdot) -> [rdot]  "rdot"
  [rdot] -> Mux/12
  MATLAB Function2/2(pdot) -> [pdot]  "pdot"
  [pdot] -> Mux/10
  MATLAB Function3/2(qdot) -> [qdot]  "qdot"
  [qdot] -> Mux/11
  MATLAB Function3/1(thetadot) -> [thetadot]  "thetadot"
  [thetadot] -> Mux/8
  MATLAB Function2/1(phidot) -> [phidot]  "phidot"
  [phidot] -> Mux/7
  [U] -> MATLAB Function2/6(U)
  [U1] -> MATLAB Function3/5(U)
  [U2] -> MATLAB Function4/6(U)
  Pulse Generator4/1 -> MATLAB Function1/5(Fy), MATLAB Function/5(Fx)

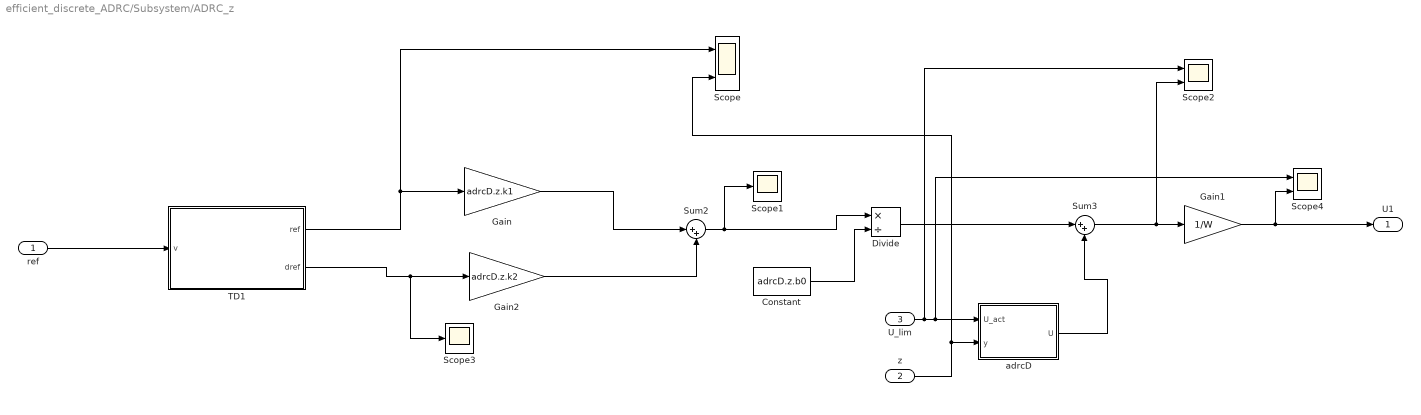
== system efficient_discrete_ADRC/Subsystem/ADRC_z ==
  ref : Inport
  z : Inport  Port=2
  U_lim : Inport  Port=3
  Constant : Constant  Value=adrcD.z.b0
  Divide : Product  Inputs=*/
  Gain : Gain  Gain=adrcD.z.k1
  Gain1 : Gain  Gain=1/W
  Gain2 : Gain  Gain=adrcD.z.k2
  Scope : Scope  NumInputPorts=2
      settings: ActiveDisplayYMinimum=-0.18629209310079653  ActiveDisplayYMaximum=1.676628837907169  DataLoggingVariableName=ScopeData24
  Scope1 : Scope
      settings: ActiveDisplayYMinimum=-1  ActiveDisplayYMaximum=1  DataLoggingVariableName=ScopeData7
  Scope2 : Scope  NumInputPorts=2
      settings: ActiveDisplayYMinimum=-22.74809658591446  ActiveDisplayYMaximum=35.265497735934922  DataLoggingVariableName=ScopeData6
  Scope3 : Scope
      settings: ActiveDisplayYMinimum=-1  ActiveDisplayYMaximum=1  DataLoggingVariableName=ScopeData12
  Scope4 : Scope  NumInputPorts=2
      settings: ActiveDisplayYMinimum=-23.663137505817438  ActiveDisplayYMaximum=40.389726887391646  DataLoggingVariableName=ScopeData5
  Sum2 : Sum  Inputs=|++
  Sum3 : Sum  Inputs=|++
  TD1 : Subsystem
  adrcD : Subsystem
  U1 : Outport
  wires:
  ref/1 -> TD1/1(v)
  TD1/1(ref) -> Gain/1, Scope/1
  Constant/1 -> Divide/2
  Gain/1 -> Sum2/1
  TD1/2(dref) -> Scope3/1, Gain2/1
  Gain2/1 -> Sum2/2
  Sum2/1 -> Scope1/1, Divide/1
  Sum3/1 -> Scope2/2, Gain1/1
  Gain1/1 -> Scope4/2, U1/1
  U_lim/1 -> Scope2/1, Scope4/1, adrcD/1(U_act)
  z/1 -> Scope/2, adrcD/2(y)
  adrcD/1(U) -> Sum3/2
  Divide/1 -> Sum3/1

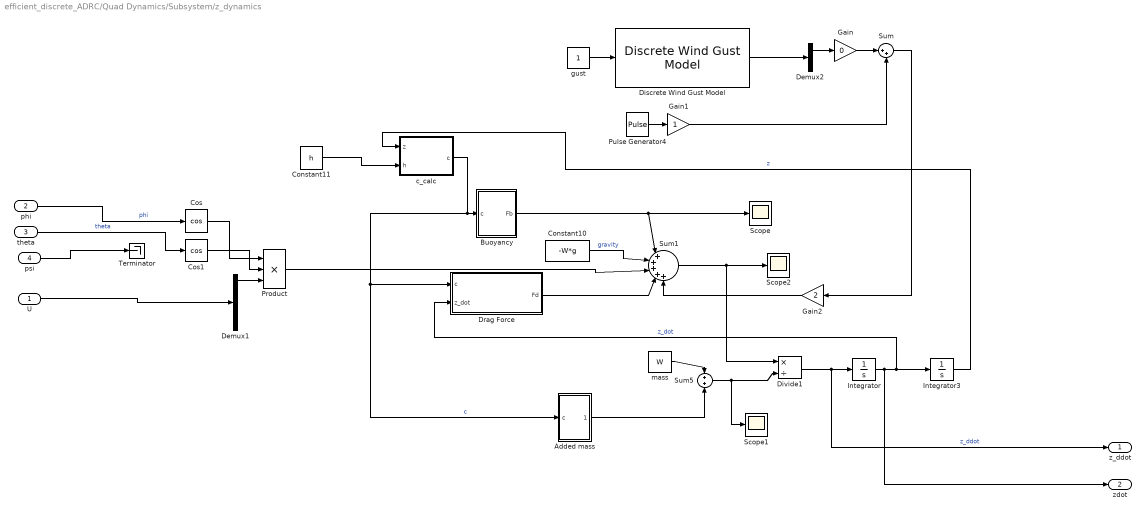
== system efficient_discrete_ADRC/Quad Dynamics/Subsystem/z_dynamics ==
  U : Inport
  phi : Inport  Port=2
  theta : Inport  Port=3
  psi : Inport  Port=4
  Added mass : Subsystem
  Buoyancy : Subsystem
  Constant10 : Constant  Value=-W*g
  Constant11 : Constant  Value=h
  Cos : Trigonometry  Operator=cos
  Cos1 : Trigonometry  Operator=cos
  Demux1 : Demux
  Demux2 : Demux  Outputs=3
  Discrete Wind Gust Model : aerolibwind2/Discrete Wind Gust Model  units=Metric (MKS)  Gx=on  Gy=off  Gz=off  t_0=7  d_m=[1 0.5 0.5]  v_m=[2 2 2]
  Divide1 : Product  Inputs=*/
  Drag Force : Subsystem
  Gain : Gain  Gain=0
  Gain1 : Gain
  Gain2 : Gain  Gain=2
  Integrator : Integrator
  Integrator3 : Integrator
  Product : Product  Inputs=3
  Pulse Generator4 : DiscretePulseGenerator  PulseType=Time based  Period=20  PulseWidth=30  PhaseDelay=5
  Scope : Scope
      settings: ActiveDisplayYMinimum=3.324205069659222  ActiveDisplayYMaximum=24.046643881148977  DataLoggingVariableName=ScopeData4
  Scope1 : Scope
      settings: ActiveDisplayYMinimum=1.2962500000000001  ActiveDisplayYMaximum=1.7337500000000001  DataLoggingVariableName=ScopeData8
  Scope2 : Scope
      settings: ActiveDisplayYMinimum=-2.7468  ActiveDisplayYMaximum=24.721200000000003  DataLoggingVariableName=ScopeData10
  Sum : Sum  Inputs=|++
  Sum1 : Sum  Inputs=|+++++
  Sum5 : Sum
  Terminator : Terminator
  c_calc : MATLAB Function  TreatAsAtomicUnit=on
  gust : Constant
  mass : Constant  Value=W
  z_ddot : Outport
  zdot : Outport  Port=2
  wires:
  phi/1 -> Cos/1  "phi"
  theta/1 -> Cos1/1  "theta"
  Cos/1 -> Product/1
  Cos1/1 -> Product/2
  Demux1/1 -> Product/3
  psi/1 -> Terminator/1
  Sum1/1 -> Scope2/1, Divide1/1
  c_calc/1(c) -> Added mass/1(c), Drag Force/1(c), Buoyancy/1(c)  "c"
  Product/1 -> Sum1/3
  Added mass/1(m_a) -> Sum5/2
  mass/1 -> Sum5/1
  Sum5/1 -> Scope1/1, Divide1/2
  Integrator3/1 -> c_calc/1(z)  "z"
  Integrator/1 -> Drag Force/2(z_dot), Integrator3/1, zdot/1  "z_dot"
  Drag Force/1(Fd) -> Sum1/4
  Divide1/1 -> z_ddot/1, Integrator/1  "z_ddot"
  Buoyancy/1(Fb) -> Sum1/1, Scope/1
  Constant10/1 -> Sum1/2  "gravity"
  Constant11/1 -> c_calc/2(h)
  U/1 -> Demux1/1
  Gain1/1 -> Sum/2
  Discrete Wind Gust Model/1 -> Demux2/1
  Demux2/1 -> Gain/1
  Gain/1 -> Sum/1
  Pulse Generator4/1 -> Gain1/1
  Sum/1 -> Gain2/1
  gust/1 -> Discrete Wind Gust Model/1
  Gain2/1 -> Sum1/5

== system efficient_discrete_ADRC/Subsystem/ADRC_z/TD1 ==
  v : Inport
  Constant11 : Constant  Value=r0_h
  Constant12 : Constant  Value=h0_h
  Delay One Step : Delay  DelayLength=1
  Delay One Step1 : Delay  DelayLength=1
  Gain3 : Gain  Gain=Ts_h
  Gain4 : Gain  Gain=Ts_h
  Sum1 : Sum  Inputs=|++
  Sum6 : Sum  Inputs=|++
  Sum7 : Sum  Inputs=|+-
  fhan : MATLAB Function  TreatAsAtomicUnit=on
  ref : Outport
  dref : Outport  Port=2
  wires:
  v/1 -> Sum7/2
  Constant12/1 -> fhan/4(h0)
  Sum7/1 -> fhan/1(e)
  Constant11/1 -> fhan/3(r0)
  Delay One Step1/1 -> fhan/2(v2), Sum6/2, Gain4/1  "v2(k)"
  Gain4/1 -> Sum1/2
  Sum1/1 -> ref/1, Delay One Step/1  "v1(k+1)"
  Sum6/1 -> dref/1, Delay One Step1/1  "v2(k+1)"
  Gain3/1 -> Sum6/1
  Delay One Step/1 -> Sum1/1, Sum7/1  "v1"
  fhan/1(u) -> Gain3/1

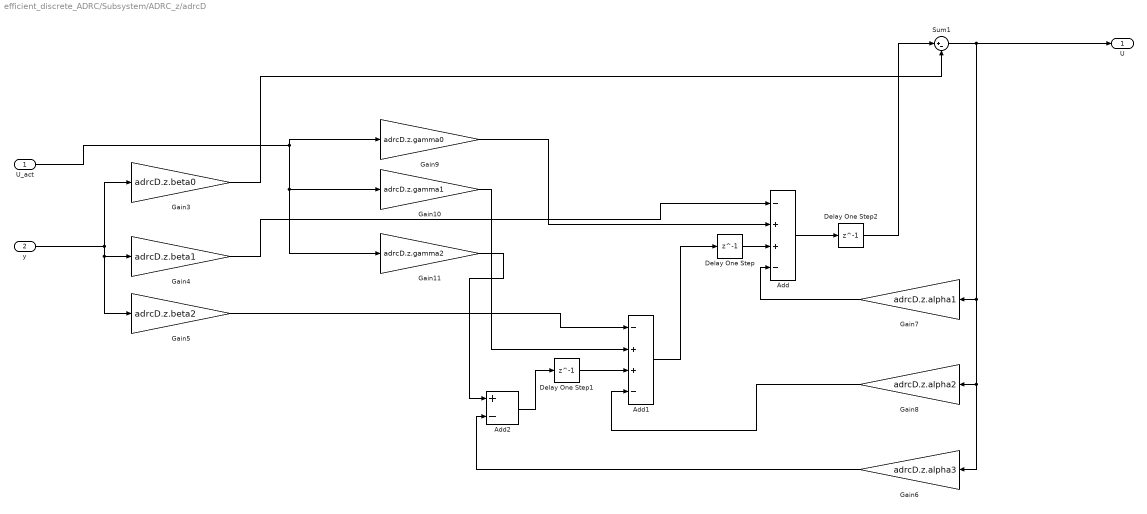
== system efficient_discrete_ADRC/Subsystem/ADRC_z/adrcD ==
  U_act : Inport
  y : Inport  Port=2
  Add : Sum  Inputs=-++-
  Add1 : Sum  Inputs=-++-
  Add2 : Sum  Inputs=+-
  Delay One Step : Delay  DelayLength=1
  Delay One Step1 : Delay  DelayLength=1
  Delay One Step2 : Delay  DelayLength=1
  Gain10 : Gain  Gain=adrcD.z.gamma1
  Gain11 : Gain  Gain=adrcD.z.gamma2
  Gain3 : Gain  Gain=adrcD.z.beta0
  Gain4 : Gain  Gain=adrcD.z.beta1
  Gain5 : Gain  Gain=adrcD.z.beta2
  Gain6 : Gain  Gain=adrcD.z.alpha3
  Gain7 : Gain  Gain=adrcD.z.alpha1
  Gain8 : Gain  Gain=adrcD.z.alpha2
  Gain9 : Gain  Gain=adrcD.z.gamma0
  Sum1 : Sum  Inputs=|+-
  U : Outport
  wires:
  Gain4/1 -> Add/1
  Gain8/1 -> Add1/4
  Add2/1 -> Delay One Step1/1
  y/1 -> Gain5/1, Gain4/1, Gain3/1
  U_act/1 -> Gain9/1, Gain11/1, Gain10/1
  Gain7/1 -> Add/4
  Gain11/1 -> Add2/1
  Gain3/1 -> Sum1/2
  Sum1/1 -> U/1, Gain6/1, Gain8/1, Gain7/1
  Add1/1 -> Delay One Step/1
  Gain5/1 -> Add1/1
  Gain10/1 -> Add1/2
  Add/1 -> Delay One Step2/1
  Gain9/1 -> Add/2
  Delay One Step1/1 -> Add1/3
  Delay One Step2/1 -> Sum1/1
  Gain6/1 -> Add2/2
  Delay One Step/1 -> Add/3

== system efficient_discrete_ADRC/Quad Dynamics/Subsystem/z_dynamics/Added mass ==
  c : Inport
  Product1 : Product
  added_mass : Constant  Value=0.05*rho_water
  m_a : Outport
  wires:
  added_mass/1 -> Product1/1
  Product1/1 -> m_a/1
  c/1 -> Product1/2

== system efficient_discrete_ADRC/Quad Dynamics/Subsystem/z_dynamics/Buoyancy ==
  c : Inport
  Constant1 : Constant  Value=rho_water*Area*g
  Product : Product
  Fb : Outport
  wires:
  Constant1/1 -> Product/2
  c/1 -> Product/1
  Product/1 -> Fb/1  "buoyancy"

== system efficient_discrete_ADRC/Quad Dynamics/Subsystem/z_dynamics/Drag Force ==
  c : Inport
  z_dot : Inport  Port=2
  Abs : Abs  SaturateOnIntegerOverflow=off
  Constant : Constant  Value=h
  Constant10 : Constant
  Constant11 : Constant  Value=Area
  Constant7 : Constant  Value=rho_air
  Constant8 : Constant  Value=rho_water
  Constant9 : Constant  Value=-0.5
  Divide : Product  Inputs=*/
  Product3 : Product
  Product4 : Product
  Product5 : Product  Inputs=5
  Sum2 : Sum
  Sum3 : Sum  Inputs=+-
  Fd : Outport
  wires:
  Divide/1 -> Sum3/2, Product4/2
  Product5/1 -> Fd/1  "drag force"
  Product4/1 -> Sum2/2  "water drag"
  Constant11/1 -> Product5/5
  Sum3/1 -> Product3/2
  Constant8/1 -> Product4/1  "water"
  Constant10/1 -> Sum3/1
  Sum2/1 -> Product5/1
  Constant9/1 -> Product5/2
  z_dot/1 -> Abs/1, Product5/3
  Abs/1 -> Product5/4
  Product3/1 -> Sum2/1  "air drag"
  Constant7/1 -> Product3/1  "air"
  c/1 -> Divide/1
  Constant/1 -> Divide/2

== matlab function efficient_discrete_ADRC/Quad Dynamics/Subsystem/z_dynamics/c_calc ==
  data: z input; c output; h input
function c = fcn(z, h)

if z > h/2
    c = 0;
elseif z < -h/2
    c = h;
else 
    c = h/2 - z;
end

== matlab function efficient_discrete_ADRC/ADRC_yaw1/TD1/fhan ==
  data: e input; u output; v2 input; r0 input; h0 input

function u = fhan(e, v2, r0, h0)

d = r0*h0^2;
a0 = h0*v2;
y = e + a0;

a1 = sqrt(d*(d + 8*abs(y)));
a2 = a0 + sign(y)*(a1 - d)/2;

sy = (sign(y + d) - sign(y - d))/2;
a = (a0 + y - a2)*sy + a2;

sa = (sign(a + d) - sign(a - d))/2;

u = -r0*(a/d - sign(a))*sa - r0*sign(a);

end

== matlab function efficient_discrete_ADRC/ADRC_roll/TD1/fhan ==
  data: e input; u output; v2 input; r0 input; h0 input

function u = fhan(e, v2, r0, h0)

d = r0*h0^2;
a0 = h0*v2;
y = e + a0;

a1 = sqrt(d*(d + 8*abs(y)));
a2 = a0 + sign(y)*(a1 - d)/2;

sy = (sign(y + d) - sign(y - d))/2;
a = (a0 + y - a2)*sy + a2;

sa = (sign(a + d) - sign(a - d))/2;

u = -r0*(a/d - sign(a))*sa - r0*sign(a);

end

== matlab function efficient_discrete_ADRC/Subsystem/ADRC_z/TD1/fhan ==
  data: e input; u output; v2 input; r0 input; h0 input

function u = fhan(e, v2, r0, h0)

d = r0*h0^2;
a0 = h0*v2;
y = e + a0;

a1 = sqrt(d*(d + 8*abs(y)));
a2 = a0 + sign(y)*(a1 - d)/2;

sy = (sign(y + d) - sign(y - d))/2;
a = (a0 + y - a2)*sy + a2;

sa = (sign(a + d) - sign(a - d))/2;

u = -r0*(a/d - sign(a))*sa - r0*sign(a);

end

== matlab function efficient_discrete_ADRC/Quad Dynamics/Subsystem/MATLAB Function ==
  data: U input; phi input; xdd output; theta input; psi input; Fx input; m input
function xdd = x_dynamics(U, phi, theta, psi, Fx, m)

T = U(1);
xdd = (T/m)*(cos(psi)*sin(theta)*cos(phi) ...
               + sin(psi)*sin(phi)) + Fx/m;

end

== matlab function efficient_discrete_ADRC/Quad Dynamics/Subsystem/MATLAB Function1 ==
  data: U input; ydd output; phi input; theta input; psi input; Fy input; m input
function ydd = y_dynamics(U, phi, theta, psi, Fy, m)

T = U(1);

ydd = (T/m)*(sin(psi)*sin(theta)*cos(phi) ...
               - cos(psi)*sin(phi)) + Fy/m;

end

== matlab function efficient_discrete_ADRC/Quad Dynamics/Subsystem/MATLAB Function2 ==
  data: phi input size=1; phidot output size=1; theta input size=1; p input size=1; q input size=1; r input size=1; U input; inertia_mx input; pdot output size=1
function [phidot, pdot] = roll_dynamics( ...
    phi, theta, p, q, r, U, inertia_mx)

Ix = inertia_mx(1);
Iy = inertia_mx(2);
Iz = inertia_mx(3);

tau_roll = U(2);

phidot = p + sin(phi)*tan(theta)*q ...
           + cos(phi)*tan(theta)*r;

pdot = (tau_roll + (Iy-Iz)*q*r)/Ix;

end

== matlab function efficient_discrete_ADRC/Quad Dynamics/Subsystem/MATLAB Function3 ==
  data: phi input size=1; thetadot output size=1; p input size=1; q input size=1; r input size=1; U input size=[4 1]; inertia_mx input size=[3 1]; qdot output size=1
function [thetadot, qdot] = pitch_dynamics( ...
    phi, p, q, r, U, inertia_mx)

Ix = inertia_mx(1);
Iy = inertia_mx(2);
Iz = inertia_mx(3);

tau_pitch = U(3);

thetadot = cos(phi)*q - sin(phi)*r;

qdot = (tau_pitch + (Iz-Ix)*p*r)/Iy;

end

== matlab function efficient_discrete_ADRC/Quad Dynamics/Subsystem/MATLAB Function4 ==
  data: phi input size=1; psidot output size=1; theta input size=1; p input size=1; q input size=1; r input size=1; U input; inertia_mx input; rdot output size=1
function [psidot, rdot] = yaw_dynamics( ...
    phi, theta, p, q, r, U, inertia_mx)

Ix = inertia_mx(1);
Iy = inertia_mx(2);
Iz = inertia_mx(3);

psidot = 0;
rdot = 0;

tau_yaw = U(4);

psidot = (sin(phi)*q + cos(phi)*r)/cos(theta);

rdot = (tau_yaw + (Ix-Iy)*p*q)/Iz;

end
